simulink model "buck_converter"  (R2025b)
settings: Solver=ode45  StartTime=0.0  StopTime=p.stopTime  MaxStep=p.sampleTime  RelTol=1e-8  AbsTol=1e-10
model workspace (MAT data in the model file):
  inputSignal = [0  24  6  0; 0.005  24  6  12; 0.00762  24  6  12; 0.00762  24  4  12; 0.01228  24  4  12; 0.01228  20  4  12; 0.01546  20  4  12]
  p.topology = 'buck'
  p.inputVoltage = 24
  p.lineVoltage = 20
  p.reference = 12
  p.startVoltage = 0
  p.resistance = 6
  p.loadedResistance = 4
  p.L = 0.0002
  p.C = 0.00022
  p.couplingCapacitance = 0.0001
  p.windingResistance = 0.04
  p.switchingFrequency = 50000
  p.currentLimit = 5
  p.maximumDuty = 0.9
  p.stateCount = 2
  p.initialState = [0; 0]
  p.initialIntegral = 0
  p.initialDutyCorrection = 0
  p.softStart = 0.005
  p.sampleTime = 2e-05
  p.sizingHorizon = 0.1
  p.loadTime = 0.00762
  p.lineTime = 0.01228
  p.stopTime = 0.01546
  p.Kpv = 1.10584061406
  p.Kiv = 1111.71223974
  p.Kpi = 0.314159265359
  p.Kii = 1184.35252813
  p.voltageTracking = 5026.54824574
  p.currentTracking = 37699.1118431
  p.modelName = 'buck_converter'
values from neighbouring files (symbols this model uses):
  p = project_parameters(); [p,timing]=plan_experiment(p)    [run_demo.m]
undefined symbols (not defined in the file or in its folder): sl_controller, sl_plant
settings Model: Creator=LENOVO  LastModifiedBy=LENOVO

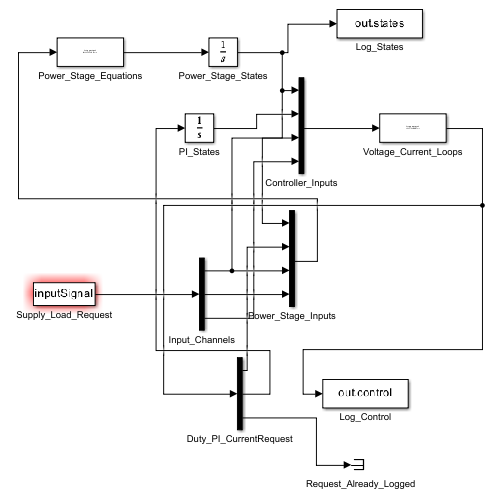
[thumbnail: Simulink's stored preview of the top-level diagram]
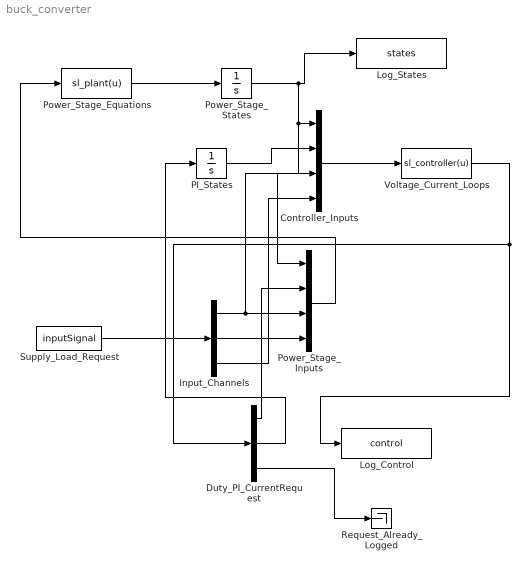
== system buck_converter ==
  Controller_Inputs : Mux
  Duty_PI_CurrentRequest : Demux  Outputs=[1 2 1]
  Input_Channels : Demux  Outputs=3
  Log_Control : ToWorkspace  VariableName=control  SaveFormat=Timeseries  SampleTime=-1
  Log_States : ToWorkspace  VariableName=states  SaveFormat=Timeseries  SampleTime=-1
  PI_States : Integrator  InitialCondition=[p.initialIntegral;p.initialDutyCorrection]
  Power_Stage_Equations : MATLABFcn  MATLABFcn=sl_plant(u)  OutputDimensions=p.stateCount
  Power_Stage_Inputs : Mux
  Power_Stage_States : Integrator  InitialCondition=p.initialState
  Request_Already_Logged : Terminator
  Supply_Load_Request : FromWorkspace  VariableName=inputSignal
  Voltage_Current_Loops : MATLABFcn  MATLABFcn=sl_controller(u)  OutputDimensions=4
  wires:
  Supply_Load_Request/1 -> Input_Channels/1
  Power_Stage_Equations/1 -> Power_Stage_States/1
  Power_Stage_Inputs/1 -> Power_Stage_Equations/1
  Voltage_Current_Loops/1 -> Log_Control/1, Duty_PI_CurrentRequest/1
  Controller_Inputs/1 -> Voltage_Current_Loops/1
  Power_Stage_States/1 -> Power_Stage_Inputs/1, Controller_Inputs/1, Log_States/1
  PI_States/1 -> Controller_Inputs/2
  Input_Channels/1 -> Power_Stage_Inputs/3, Controller_Inputs/3
  Input_Channels/3 -> Controller_Inputs/4
  Duty_PI_CurrentRequest/2 -> PI_States/1
  Duty_PI_CurrentRequest/3 -> Request_Already_Logged/1
  Duty_PI_CurrentRequest/1 -> Power_Stage_Inputs/2
  Input_Channels/2 -> Power_Stage_Inputs/4
